simulink model "AFC_FFNN_trainlm_45_45_45_Nor_July_15"  (R2021a)
settings: Solver=ode15s  StartTime=0.0  StopTime=T  MaxStep=.01  RelTol=1e-3
undefined symbols (not defined in the file): AF_sensor_tol, fault_time, fuel_inj_tol, kappa_tol, MAF_sensor_tol, pump_tol, tau_ww_tol, x_gain, x_offset, y_gain, y_offset
libraries: neural x140
(part 6 of 6)

== system AFC_FFNN_trainlm_45_45_45_Nor_July_15/Air Fuel Control Model 1/Feed-Forward Neural Network/Layer 4/Delays 1 ==
  "p{4}" : Inport  PortDimensions=45
      mask Display: e = 0.06;c1 = [120 230 180]/255;c2 = ([120 230 180]+0)/(256+128);c3 = ([120 230 180]+128)/(256+128);patch([0 1 1 0],[0 0 1 1],c1);patch([0 1 1 1-e 1-e 0+e],[0 0 1 1-e 0+e 0+e],c2);patch([0 0 1 1-e 0+e 0+e],[0 1 1 1-e 1-e 0+e],c3);plot([0 1 1 0 0],[0 0 1 1 0]);
  mux : Mux  Inputs=1
      mask Display: e = 0.06;c1 = [120 150 230]/255;c2 = ([120 150 230]+0)/383;c3 = ([120 150 230]+128)/383;patch([0 1 1 0],[0 0 1 1],c1);patch([0 1 1 1-e 1-e 0+e],[0 0 1 1-e 0+e 0+e],c2);patch([0 0 1 1-e 0+e 0+e],[0 1 1 1-e 1-e 0+e],c3);plot([0 1 1 0 0],[0 0 1 1 0]);disp('Mux')
  "pd{4,3}" : Outport
      mask Display: e = 0.06;c1 = [120 230 180]/255;c2 = ([120 230 180]+0)/(256+128);c3 = ([120 230 180]+128)/(256+128);patch([0 1 1 0],[0 0 1 1],c1);patch([0 1 1 1-e 1-e 0+e],[0 0 1 1-e 0+e 0+e],c2);patch([0 0 1 1-e 0+e 0+e],[0 1 1 1-e 1-e 0+e],c3);plot([0 1 1 0 0],[0 0 1 1 0]);
  wires:
  mux/1 -> "pd{4,3}"/1
  "p{4}"/1 -> mux/1

== system AFC_FFNN_trainlm_45_45_45_Nor_July_15/Air Fuel Control Model 1/Feed-Forward Neural Network/Layer 4/LW{4,3} ==
  "ad{4,3}" : Inport  PortDimensions=45
      mask Display: e = 0.06;c1 = [120 230 180]/255;c2 = ([120 230 180]+0)/(256+128);c3 = ([120 230 180]+128)/(256+128);patch([0 1 1 0],[0 0 1 1],c1);patch([0 1 1 1-e 1-e 0+e],[0 0 1 1-e 0+e 0+e],c2);patch([0 0 1 1-e 0+e 0+e],[0 1 1 1-e 1-e 0+e],c3);plot([0 1 1 0 0],[0 0 1 1 0]);
  "IW{4,3}(1,:)'" : Constant  Value=[0.8109570338987313053991101696738041937351226806640625;-0.124727127087947808892209877740242518484592437744140625;-0.231351350840265646002791299906675703823566436767578125;0.0296658340037450340975766494011622853577136993408203125;-0.1584122531555937352099050485776388086378574371337890625;-0.42466520306568877884956236812286078929901123046875;0.46852473737176281165517366389394737780094146728515625;-0.144975282849131748008630893309600651264190673828125;0.011230631725688451638678344579602708108723163604736328125;-0.0701076693478557277927620816626586019992828369140625;0.1983118701026646280016763057574280537664890289306640625;-0.7527867532732204214340754333534277975559234619140625;0.121895216825640695379462385972146876156330108642578125;0.0199954344692183615117553330264854594133794307708740234375;0.97773336297479540579757895102375186979770660400390625;-0.057695952177792990400728712074851500801742076873779296875;-0.0997373888236172678745106168207712471485137939453125;0.005054455996690379766811407336035699700005352497100830078125;-0.007241885173675895702449789581578443176113069057464599609375;-0.6993076111322731325259383083903230726718902587890625;0.064779107847705630351953232093364931643009185791015625;-0.0106077365330169183510466979214470484293997287750244140625;0.3768577374736263863042040611617267131805419921875;0.01494103413290641564625804704746769857592880725860595703125;-0.042680769327031777005121426782352500595152378082275390625;-0.0193281614750664028357096668742087786085903644561767578125;0.2476028183430607487736097027664072811603546142578125;0.00074855081871878152537103101593629617127589881420135498046875;-0.09853924414225366523734095380859798751771450042724609375;-0.82567749482011709716289260541088879108428955078125;-0.045776836705528574367196625871656578965485095977783203125;-0.2023759759360867216404500368298613466322422027587890625;-0.155970765168726099858531597419641911983489990234375;0.036563574006282385797650391623392351903021335601806640625;-0.04325115650910534015327613133194972760975360870361328125;0.059302412047336668099450918134607491083443164825439453125;0.02260032156229709043859799066922278143465518951416015625;-0.01066759310756866009628485159055344411171972751617431640625;-0.6319165389924723541525963810272514820098876953125;0.267416748871924514485698409771430306136608123779296875;-0.953634341950244657226676281425170600414276123046875;-0.056784119970184905590304680345070664770901203155517578125;-0.5392334952110300339001014435780234634876251220703125;0.06949610093794698906233264779075398109853267669677734375;-0.213847216262530726016422022439655847847461700439453125]
      mask Display: e = 0.06;c1 = [120 150 230]/255;c2 = ([120 150 230]+0)/383;c3 = ([120 150 230]+128)/383;patch([0 1 1 0],[0 0 1 1],c1);patch([0 1 1 1-e 1-e 0+e],[0 0 1 1-e 0+e 0+e],c2);patch([0 0 1 1-e 0+e 0+e],[0 1 1 1-e 1-e 0+e],c3);plot([0 1 1 0 0],[0 0 1 1 0]);disp('weights');
  Mux : Mux  Inputs=1
      mask Display: e = 0.06;c1 = [120 150 230]/255;c2 = ([120 150 230]+0)/383;c3 = ([120 150 230]+128)/383;patch([0 1 1 0],[0 0 1 1],c1);patch([0 1 1 1-e 1-e 0+e],[0 0 1 1-e 0+e 0+e],c2);patch([0 0 1 1-e 0+e 0+e],[0 1 1 1-e 1-e 0+e],c3);plot([0 1 1 0 0],[0 0 1 1 0]);disp('Mux');
  dotprod1 : neural/Weight Functions/dotprod
  "lz{4,3}" : Outport
      mask Display: e = 0.06;c1 = [120 230 180]/255;c2 = ([120 230 180]+0)/(256+128);c3 = ([120 230 180]+128)/(256+128);patch([0 1 1 0],[0 0 1 1],c1);patch([0 1 1 1-e 1-e 0+e],[0 0 1 1-e 0+e 0+e],c2);patch([0 0 1 1-e 0+e 0+e],[0 1 1 1-e 1-e 0+e],c3);plot([0 1 1 0 0],[0 0 1 1 0]);
  wires:
  Mux/1 -> "lz{4,3}"/1
  dotprod1/1 -> Mux/1
  "ad{4,3}"/1 -> dotprod1/2
  "IW{4,3}(1,:)'"/1 -> dotprod1/1
